simulink model "demo_cpi"  (R2026a)
settings: Solver=FixedStepAuto  StopTime=2  FixedStep=0.00025
libraries: mfeval_LIB x1
Description:
  | Copyright 2020-2024 The MathWorks, Inc.
settings Model: Creator=MFURLANT  LastModifiedBy=andrei

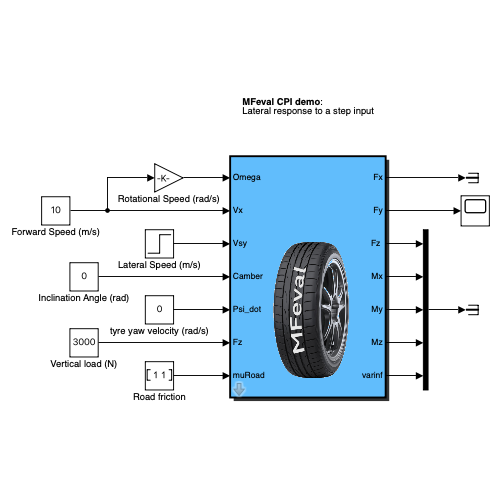
[thumbnail: Simulink's stored preview of the top-level diagram]
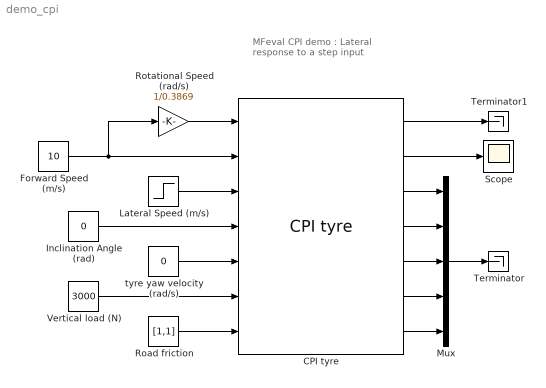
== system demo_cpi ==
  note: MFeval CPI demo :
      | Lateral response to a step input
  CPI tyre : mfeval_LIB/CPI tyre  Description=Magic Formula 6.1.2 tyre model including relaxation length and transient calculations  userParameterSource='MagicFormula61_Paramerters.tir'  userSide=1 left  userDynamics=2 linear transients  userUseMode=1 combined  enablePressure=off  userPressure=2.3
      settings: SourceProductName=MFeval Library
  Forward Speed (m/s) : Constant  Value=10
  Inclination Angle (rad) : Constant  Value=0
  Lateral Speed (m/s) : Step  SampleTime=0
  Mux : Mux  Inputs=5
  Road friction : Constant  Value=[1,1]
  Rotational Speed (rad/s) : Gain  Gain=1/0.3869
  Scope : Scope
      settings: ActiveDisplayYMinimum=-3639.8016  ActiveDisplayYMaximum=470.58715
  Terminator : Terminator
  Terminator1 : Terminator
  Vertical load (N) : Constant  Value=3000
  tyre yaw velocity (rad/s) : Constant  Value=0
  wires:
  Forward Speed (m/s)/1 -> Rotational Speed (rad/s)/1, CPI tyre/2
  Lateral Speed (m/s)/1 -> CPI tyre/3
  Inclination Angle (rad)/1 -> CPI tyre/4
  tyre yaw velocity (rad/s)/1 -> CPI tyre/5
  Vertical load (N)/1 -> CPI tyre/6
  Rotational Speed (rad/s)/1 -> CPI tyre/1
  CPI tyre/6 -> Mux/4
  CPI tyre/5 -> Mux/3
  CPI tyre/4 -> Mux/2
  CPI tyre/3 -> Mux/1
  Mux/1 -> Terminator/1
  CPI tyre/1 -> Terminator1/1
  CPI tyre/7 -> Mux/5
  CPI tyre/2 -> Scope/1
  Road friction/1 -> CPI tyre/7
